simulink model "SimuLift_WithAnimation"  (R2025b)
settings: Solver=VariableStepAuto  StartTime=0.0  StopTime=10.0  RelTol=1e-3
libraries: simulink x3
settings Model: Creator=Utente  LastModifiedBy=Utente

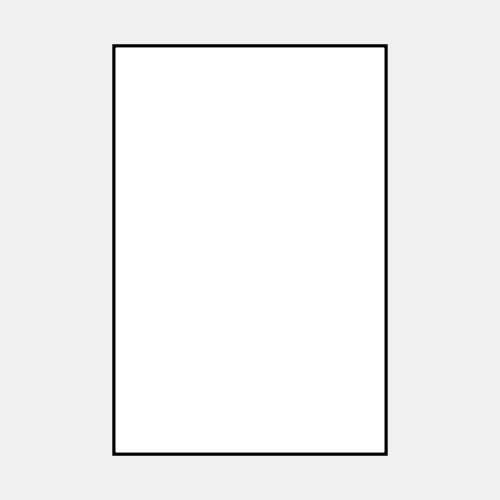
[thumbnail: Simulink's stored preview of the top-level diagram]
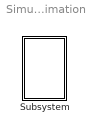
== system SimuLift_WithAnimation ==
  Subsystem : Subsystem

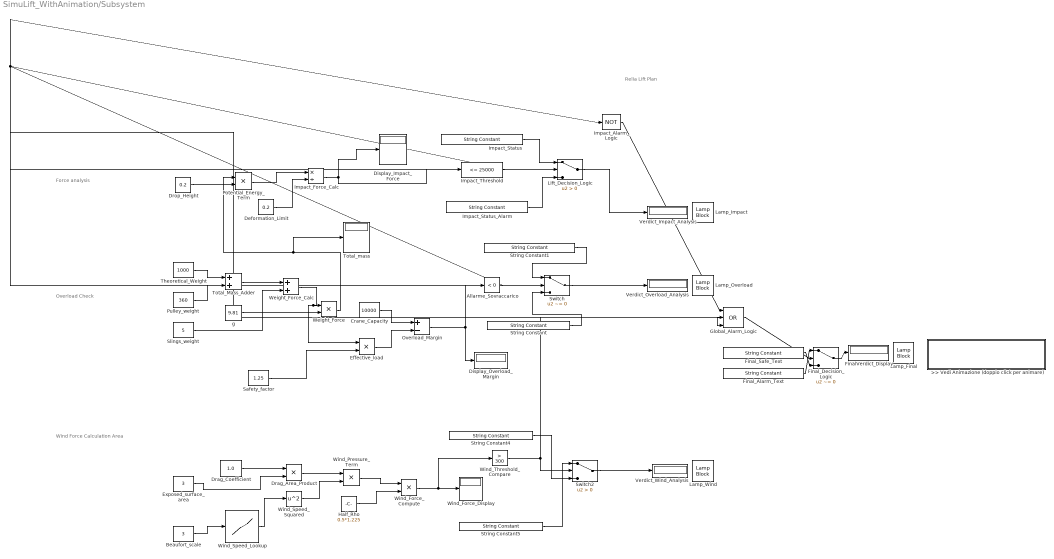
== system SimuLift_WithAnimation/Subsystem ==
  note: Force analysis
  note: Relia Lift Plan
  note: Wind Force Calculation Area
  note: Overload Check
  >> Vedi Animazione (doppio click per animare) : Subsystem
      settings: OpenFcn=mdlPath = fileparts(get_param(bdroot,'FileName')); if isempty(mdlPath), mdlPath = pwd; end; addpath(mdlPath); xlsxPath = fullfile(mdlPath, 'SimuLift_Dati_Sollevamento.xlsx'); if ~isfile(xlsxPath), xlsxPath = 'SimuLift_Dati_Sollevamento.xlsx'; end; simulift_animate_2d(xlsxPath, false);
  Allarme_Sovraccarico : simulink/Logic and Bit Operations/Compare To Zero  relop=<  OutDataTypeStr=boolean
  Beaufort_scale : Constant  Value=3
  Crane_Capacity : Constant  Value=10000
  Deformation_Limit : Constant  Value=0.2
  Display_Impact_Force : Display
      settings: Format=bank
  Display_Overload_Margin : Display
      settings: Format=bank
  Drag_Area_Product : Product
  Drag_Coefficient : Constant  Value=1.0
  Drop_Height : Constant  Value=0.2
  Effective_load : Product
  Exposed_surface_area : Constant  Value=3
  FinalVerdict_Display : Display
  Final_Alarm_Text : StringConstant  String="\"LIFT DENIED\""
  Final_Decision_Logic : Switch  Criteria=u2 ~= 0  SaturateOnIntegerOverflow=off  InputSameDT=off
  Final_Safe_Text : StringConstant  String="\"SAFE TO LIFT\""
  Global_Alarm_Logic : Logic  Operator=OR  Inputs=3
  Half_Rho : Constant  Value=0.5*1.225
  Impact_Alarm_Logic : Logic  Operator=NOT
  Impact_Force_Calc : Product  Inputs=*/
  Impact_Status : StringConstant  String="\"Safe To Lift\""
  Impact_Status_Alarm : StringConstant  String="\"impact_Force_Alarm\""
  Impact_Threshold : simulink/Logic and Bit Operations/Compare To Constant  relop=<=  const=25000  OutDataTypeStr=boolean
  Lamp_Final : LampBlock  LabelPosition=Hide  DefaultColor=[192.0, 192.0, 192.0]
  Lamp_Impact : LampBlock  LabelPosition=Hide  DefaultColor=[192.0, 192.0, 192.0]
  Lamp_Overload : LampBlock  LabelPosition=Hide  DefaultColor=[192.0, 192.0, 192.0]
  Lamp_Wind : LampBlock  LabelPosition=Hide  DefaultColor=[192.0, 192.0, 192.0]
  Lift_Decision_Logic : Switch  Criteria=u2 > Threshold  SaturateOnIntegerOverflow=off  InputSameDT=off
  Overload_Margin : Sum  Inputs=+-
  Potential_Energy_Term : Product
  Pulley_weight : Constant  Value=360
  Safety_factor : Constant  Value=1.25
  Slings_weight : Constant  Value=5
  String Constant : StringConstant  String="\"Safe To Lift\""
  String Constant1 : StringConstant  String="\"Overload Alarm\""
  String Constant4 : StringConstant  String="\"Safe To Lift\""
  String Constant5 : StringConstant  String="\"Wind_Alarm\""
  Switch : Switch  Criteria=u2 ~= 0  SaturateOnIntegerOverflow=off  InputSameDT=off
  Switch2 : Switch  Criteria=u2 > Threshold  SaturateOnIntegerOverflow=off  InputSameDT=off
  Theoretical_Weight : Constant  Value=1000
  Total_Mass_Adder : Sum
  Total_mass : Display
      settings: Format=bank
  Verdict_Impact_Analysis : Display
  Verdict_Overload_Analysis : Display
  Verdict_Wind_Analysis : Display
      settings: Format=bank
  Weight_Force : Product
  Weight_Force_Calc : Sum
  Wind_Force_Compute : Product
  Wind_Force_Display : Display
  Wind_Pressure_Term : Product
  Wind_Speed_Lookup : Lookup_n-D  NumberOfTableDimensions=1  BreakpointsForDimension1=[0;1;2;3;4;5;6;7;9;10;11;12]  Table=[0;1.5;3.2999999999999998;5.4000000000000004;7.9000000000000004;10.699999999999999;13.800000000000001;17.100000000000001;20.699999999999999;24.399999999999999;28.399999999999999;36.899999999999999]  InternalRulePriority=Speed  RndMeth=Simplest
  Wind_Speed_Squared : Math  Operator=square
  Wind_Threshold_Compare : simulink/Logic and Bit Operations/Compare To Constant  relop=>  const=300  OutDataTypeStr=boolean
  g : Constant  Value=9.81
  wires:
  Drop_Height/1 -> Potential_Energy_Term/2
  Wind_Force_Compute/1 -> Wind_Threshold_Compare/1, Wind_Force_Display/1
  Slings_weight/1 -> Weight_Force_Calc/2
  Wind_Speed_Lookup/1 -> Wind_Speed_Squared/1
  Wind_Threshold_Compare/1 -> Switch2/2, Global_Alarm_Logic/3
  Drag_Area_Product/1 -> Wind_Pressure_Term/1
  Impact_Force_Calc/1 -> Display_Impact_Force/1, Impact_Threshold/1
  Drag_Coefficient/1 -> Drag_Area_Product/1
  Potential_Energy_Term/1 -> Impact_Force_Calc/1
  Deformation_Limit/1 -> Impact_Force_Calc/2
  String Constant5/1 -> Switch2/1
  g/1 -> Weight_Force/2
  Impact_Status_Alarm/1 -> Lift_Decision_Logic/3
  Exposed_surface_area/1 -> Drag_Area_Product/2
  Overload_Margin/1 -> Allarme_Sovraccarico/1, Display_Overload_Margin/1
  Wind_Pressure_Term/1 -> Wind_Force_Compute/1
  Weight_Force_Calc/1 -> Effective_load/1, Weight_Force/1
  Theoretical_Weight/1 -> Total_Mass_Adder/1
  String Constant1/1 -> Switch/1
  Beaufort_scale/1 -> Wind_Speed_Lookup/1
  Weight_Force/1 -> Potential_Energy_Term/1, Total_mass/1
  Effective_load/1 -> Overload_Margin/2
  Allarme_Sovraccarico/1 -> Switch/2, Global_Alarm_Logic/2
  Wind_Speed_Squared/1 -> Wind_Pressure_Term/2
  Lift_Decision_Logic/1 -> Verdict_Impact_Analysis/1
  Switch2/1 -> Verdict_Wind_Analysis/1
  Half_Rho/1 -> Wind_Force_Compute/2
  Switch/1 -> Verdict_Overload_Analysis/1
  Pulley_weight/1 -> Total_Mass_Adder/2
  String Constant/1 -> Switch/3
  Safety_factor/1 -> Effective_load/2
  Impact_Threshold/1 -> Lift_Decision_Logic/2, Impact_Alarm_Logic/1
  Impact_Status/1 -> Lift_Decision_Logic/1
  Total_Mass_Adder/1 -> Weight_Force_Calc/1
  String Constant4/1 -> Switch2/3
  Crane_Capacity/1 -> Overload_Margin/1
  Impact_Alarm_Logic/1 -> Global_Alarm_Logic/1
  Global_Alarm_Logic/1 -> Final_Decision_Logic/2
  Final_Safe_Text/1 -> Final_Decision_Logic/3
  Final_Alarm_Text/1 -> Final_Decision_Logic/1
  Final_Decision_Logic/1 -> FinalVerdict_Display/1

== system SimuLift_WithAnimation/Subsystem/>> Vedi Animazione (doppio click per animare) ==
  wires:
  ? -> ?
